simulink model "BLDC_simulator"  (R2024a)
settings: Solver=ode4  StartTime=0.0  StopTime=T  MaxStep=20e-5  RelTol=1e-3  EnableMultiTasking=on
PreLoadFcn:
  | % load scdfocmotorPIDTuning_initial
  | % set_parameters
values from neighbouring files (symbols this model uses):
  current_loop = 1    [BLDC_simulator_init_control.m]    (also in BLDC_simulator_init_control_net_v2_stats_multi.m)
  i_omega = 2.497  * coeff(rand())    [set_parameters_perturbed.m]
  paramPwmCompareAtZeroVolt = 330    [set_parameters_perturbed.m]
  paramPwmCompareMax = 660    [set_parameters_perturbed.m]
  paramPwmComparePerVolt = paramPwmCompareMax/2/BLDC.RatedVoltage    [set_parameters_perturbed.m]
  speed_loop = 1    [BLDC_simulator_init_control.m]    (also in BLDC_simulator_init_control_net_v2_stats_multi.m)
undefined symbols (not defined in the file or in its folder): BLDC, inverter, PID_current, PID_speed, pwm, sampleTime
libraries: nesl_utility x13, fl_lib x12, ee_lib x8, slpidlib x3, simulink x1
(part 2 of 2)

== system BLDC_simulator/Motor_And_Load/Voltage_To_PWM_Compare ==
  note: Voltage To PWM Compare
  Voltage : Inport
  Add : Sum  OutDataTypeStr=Inherit: Inherit via back propagation
  Bias : Constant  Value=paramPwmCompareAtZeroVolt  OutDataTypeStr=Inherit: Inherit via back propagation  SampleTime=-1
  Data_Type_Conversion : DataTypeConversion  OutDataTypeStr=uint16  SaturateOnIntegerOverflow=off  RndMeth=Floor  LockScale=on
  Saturation : Saturate  UpperLimit=paramPwmCompareMax  LowerLimit=0
      settings: AttributesFormatString=|
      | --------------------------------
      | Upper Limit = %<UpperLimit>
      | Lower Limit = %<LowerLimit>
  Slope : Gain  Gain=paramPwmComparePerVolt
      settings: AttributesFormatString=|
      | ----------------------------------------
      | Gain = %<Gain>
  Compare : Outport  VectorParamsAs1DForOutWhenUnconnected=off
  wires:
  Data_Type_Conversion/1 -> Compare/1  "pwmCompare"
  Voltage/1 -> Slope/1  "phaseVoltage"
  Slope/1 -> Add/1
  Saturation/1 -> Data_Type_Conversion/1
  Bias/1 -> Add/2
  Add/1 -> Saturation/1

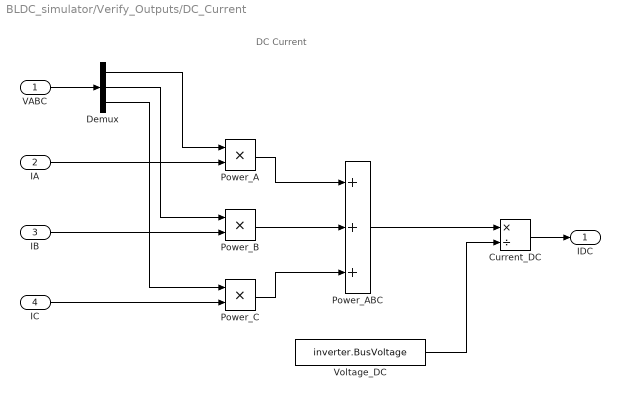
== system BLDC_simulator/Verify_Outputs/DC_Current ==
  note: DC Current
  VABC : Inport
  IA : Inport  Port=2
  IB : Inport  Port=3
  IC : Inport  Port=4
  Current_DC : Product  Inputs=*/
  Demux : Demux  Outputs=3
  Power_A : Product
  Power_ABC : Sum  Inputs=+++
  Power_B : Product
  Power_C : Product
  Voltage_DC : Constant  Value=inverter.BusVoltage
  IDC : Outport  VectorParamsAs1DForOutWhenUnconnected=off
  wires:
  Demux/3 -> Power_C/1
  Demux/2 -> Power_B/1
  Demux/1 -> Power_A/1
  IC/1 -> Power_C/2
  IB/1 -> Power_B/2
  IA/1 -> Power_A/2
  Power_ABC/1 -> Current_DC/1
  Voltage_DC/1 -> Current_DC/2
  Current_DC/1 -> IDC/1
  Power_C/1 -> Power_ABC/3
  VABC/1 -> Demux/1
  Power_B/1 -> Power_ABC/2
  Power_A/1 -> Power_ABC/1

== system BLDC_simulator/Controller_Algorithm/DQ_Current_Control/D_Current_Control ==
  note: D Current Control
  note: D Current Control
  Current_Command : Inport
  Current_Measured : Inport  Port=2
  D current Scope : Scope  NumInputPorts=2
  Error : Sum  Inputs=+-
  PI Controller : slpidlib/PID Controller  Controller=PI  Form=Parallel  TimeDomain=Discrete-time  UseExternalTs=off  SampleTime=sampleTime.CurrentControl  IntegratorMethod=Forward Euler  FilterMethod=Forward Euler  ControllerParametersSource=internal  P=PID_current.p  I=PID_current.i  UseKiTs=off  D=5e-5  UseExternalDerivativeSource=off  N=20000  UseFilter=off  TunerSelectOption=Frequency Response Based  InitialConditionSource=internal  InitialConditionForIntegrator=0  InitialConditionForFilter=0  DifferentiatorICPrevScaledInput=0  ExternalReset=none  TrackingMode=off  Kt=1  LimitOutput=on  SatLimitsSource=internal  UpperSaturationLimit=BLDC.VoltageMax  LowerSaturationLimit=-BLDC.VoltageMax  LinearizeAsGain=off  AntiWindupMode=clamping  Kb=100  LimitIntegrator=off  UpperIntegratorSaturationLimit=inf  LowerIntegratorSaturationLimit=-inf  POutMin=[]  POutMax=[]  IOutMin=[]  IOutMax=[]  DOutMin=[]  DOutMax=[]  NOutMin=[]  NOutMax=[]  SumOutMin=[]  SumOutMax=[]  SaturationOutMin=[]  SaturationOutMax=[]  PParamMin=[]  PParamMax=[]  IParamMin=[]  IParamMax=[]  DParamMin=[]  DParamMax=[]  NParamMin=[]  NParamMax=[]  KbParamMin=[]  KbParamMax=[]  KtParamMin=[]  KtParamMax=[]  KbOutMin=[]  KbOutMax=[]  KtOutMin=[]  KtOutMax=[]  IntegratorOutMin=[]  IntegratorOutMax=[]  FilterOutMin=[]  FilterOutMax=[]  SumI1OutMin=[]  SumI1OutMax=[]  SumI2OutMin=[]  SumI2OutMax=[]  SumI3OutMin=[]  SumI3OutMax=[]  SumI4OutMin=[]  SumI4OutMax=[]  SumDOutMin=[]  SumDOutMax=[]  DifferentiatorOutMin=[]  DifferentiatorOutMax=[]  FilterDiffOutCoefMin=[]  FilterDiffOutCoefMax=[]  ReciprocalOutMin=[]  ReciprocalOutMax=[]  SumDenOutMin=[]  SumDenOutMax=[]  SumNumOutMin=[]  SumNumOutMax=[]  DivideOutMin=[]  DivideOutMax=[]  UdiffTsProdOutMin=[]  UdiffTsProdOutMax=[]  NTsProdOutMin=[]  NTsProdOutMax=[]  UintegralTsProdOutMin=[]  UintegralTsProdOutMax=[]  UngainTsProdOutMin=[]  UngainTsProdOutMax=[]  ClampingZeroOutDataTypeStr=Inherit: Inherit via back propagation  ClampingZeroOutMin=[]  ClampingZeroOutMax=[]  FilterDenConstantOutDataTypeStr=Inherit: Inherit via back propagation  FilterDenConstantOutMin=[]  FilterDenConstantOutMax=[]  PCopyOutDataTypeStr=Inherit: Inherit via back propagation  PCopyOutMin=[]  PCopyOutMax=[]  NCopyOutDataTypeStr=Inherit: Inherit via back propagation  NCopyOutMin=[]  NCopyOutMax=[]  IntegratorContinuousStateAttributes=''  IntegratorStateMustResolveToSignalObject=off  IntegratorRTWStateStorageClass=Auto  FilterContinuousStateAttributes=''  FilterStateMustResolveToSignalObject=off  FilterRTWStateStorageClass=Auto  ParallelPVariant=InternalParameters  IdealPVariant=Disabled  IVariant=InternalParameters  DVariant=Disabled  IntegratorVariant=Discrete  SatVariant=Enabled  AWVariant=DiscClampingParallel  PCopyVariant=Disabled  TRVariant=Disabled  FdbkBlocksVariant=Forward  IdealPFdbkVariant=Disabled  SatFdbkVariant=Disabled  DerivativeFilterVariant=Disabled  NVariant=Disabled  NCopyVariant=Disabled_SignalSpec  FilterICVariant=Disabled  IntegratorICVariant=InternalICs  ExternalResetVariant=Disabled  TRSumVariant=Passthrough  SumFdbkVariant=Disabled  SumVariant=Sum_PI  TsampFilterVariant=InternalTs  TsampNgainVariant=Passthrough  TsampIntegralVariant=Disabled_SignalSpec  ExternalSaturationOutDataTypeStr=Inherit: Same as second input  DerivativeSourceVariant=Disabled
  Voltage : Outport  VectorParamsAs1DForOutWhenUnconnected=off
  wires:
  Error/1 -> PI Controller/1  "currentControlError"
  Current_Command/1 -> Error/1
  PI Controller/1 -> Voltage/1, D current Scope/1  "voltage"
  Current_Measured/1 -> Error/2, D current Scope/2  "current"

== system BLDC_simulator/Controller_Algorithm/DQ_Current_Control/Q_Current_Control ==
  note: Q Current Control
  note: Q Current Control
  Current_Command : Inport
  Current_Measured : Inport  Port=2
  D current Scope : Scope  NumInputPorts=2
  Error : Sum  Inputs=+-
  PI Controller : slpidlib/PID Controller  Controller=PI  Form=Parallel  TimeDomain=Discrete-time  UseExternalTs=off  SampleTime=sampleTime.CurrentControl  IntegratorMethod=Forward Euler  FilterMethod=Forward Euler  ControllerParametersSource=internal  P=PID_current.p  I=PID_current.i  UseKiTs=off  D=5e-5  UseExternalDerivativeSource=off  N=20000  UseFilter=off  TunerSelectOption=Frequency Response Based  InitialConditionSource=internal  InitialConditionForIntegrator=0  InitialConditionForFilter=0  DifferentiatorICPrevScaledInput=0  ExternalReset=none  TrackingMode=off  Kt=1  LimitOutput=on  SatLimitsSource=internal  UpperSaturationLimit=BLDC.VoltageMax  LowerSaturationLimit=-BLDC.VoltageMax  LinearizeAsGain=off  AntiWindupMode=clamping  Kb=100  LimitIntegrator=off  UpperIntegratorSaturationLimit=inf  LowerIntegratorSaturationLimit=-inf  POutMin=[]  POutMax=[]  IOutMin=[]  IOutMax=[]  DOutMin=[]  DOutMax=[]  NOutMin=[]  NOutMax=[]  SumOutMin=[]  SumOutMax=[]  SaturationOutMin=[]  SaturationOutMax=[]  PParamMin=[]  PParamMax=[]  IParamMin=[]  IParamMax=[]  DParamMin=[]  DParamMax=[]  NParamMin=[]  NParamMax=[]  KbParamMin=[]  KbParamMax=[]  KtParamMin=[]  KtParamMax=[]  KbOutMin=[]  KbOutMax=[]  KtOutMin=[]  KtOutMax=[]  IntegratorOutMin=[]  IntegratorOutMax=[]  FilterOutMin=[]  FilterOutMax=[]  SumI1OutMin=[]  SumI1OutMax=[]  SumI2OutMin=[]  SumI2OutMax=[]  SumI3OutMin=[]  SumI3OutMax=[]  SumI4OutMin=[]  SumI4OutMax=[]  SumDOutMin=[]  SumDOutMax=[]  DifferentiatorOutMin=[]  DifferentiatorOutMax=[]  FilterDiffOutCoefMin=[]  FilterDiffOutCoefMax=[]  ReciprocalOutMin=[]  ReciprocalOutMax=[]  SumDenOutMin=[]  SumDenOutMax=[]  SumNumOutMin=[]  SumNumOutMax=[]  DivideOutMin=[]  DivideOutMax=[]  UdiffTsProdOutMin=[]  UdiffTsProdOutMax=[]  NTsProdOutMin=[]  NTsProdOutMax=[]  UintegralTsProdOutMin=[]  UintegralTsProdOutMax=[]  UngainTsProdOutMin=[]  UngainTsProdOutMax=[]  ClampingZeroOutDataTypeStr=Inherit: Inherit via back propagation  ClampingZeroOutMin=[]  ClampingZeroOutMax=[]  FilterDenConstantOutDataTypeStr=Inherit: Inherit via back propagation  FilterDenConstantOutMin=[]  FilterDenConstantOutMax=[]  PCopyOutDataTypeStr=Inherit: Inherit via back propagation  PCopyOutMin=[]  PCopyOutMax=[]  NCopyOutDataTypeStr=Inherit: Inherit via back propagation  NCopyOutMin=[]  NCopyOutMax=[]  IntegratorContinuousStateAttributes=''  IntegratorStateMustResolveToSignalObject=off  IntegratorRTWStateStorageClass=Auto  FilterContinuousStateAttributes=''  FilterStateMustResolveToSignalObject=off  FilterRTWStateStorageClass=Auto  ParallelPVariant=InternalParameters  IdealPVariant=Disabled  IVariant=InternalParameters  DVariant=Disabled  IntegratorVariant=Discrete  SatVariant=Enabled  AWVariant=DiscClampingParallel  PCopyVariant=Disabled  TRVariant=Disabled  FdbkBlocksVariant=Forward  IdealPFdbkVariant=Disabled  SatFdbkVariant=Disabled  DerivativeFilterVariant=Disabled  NVariant=Disabled  NCopyVariant=Disabled_SignalSpec  FilterICVariant=Disabled  IntegratorICVariant=InternalICs  ExternalResetVariant=Disabled  TRSumVariant=Passthrough  SumFdbkVariant=Disabled  SumVariant=Sum_PI  TsampFilterVariant=InternalTs  TsampNgainVariant=Passthrough  TsampIntegralVariant=Disabled_SignalSpec  ExternalSaturationOutDataTypeStr=Inherit: Same as second input  DerivativeSourceVariant=Disabled
  Voltage : Outport  VectorParamsAs1DForOutWhenUnconnected=off
  wires:
  Error/1 -> PI Controller/1  "currentControlError"
  Current_Command/1 -> Error/1
  PI Controller/1 -> Voltage/1, D current Scope/1  "voltage"
  Current_Measured/1 -> Error/2, D current Scope/2  "current"

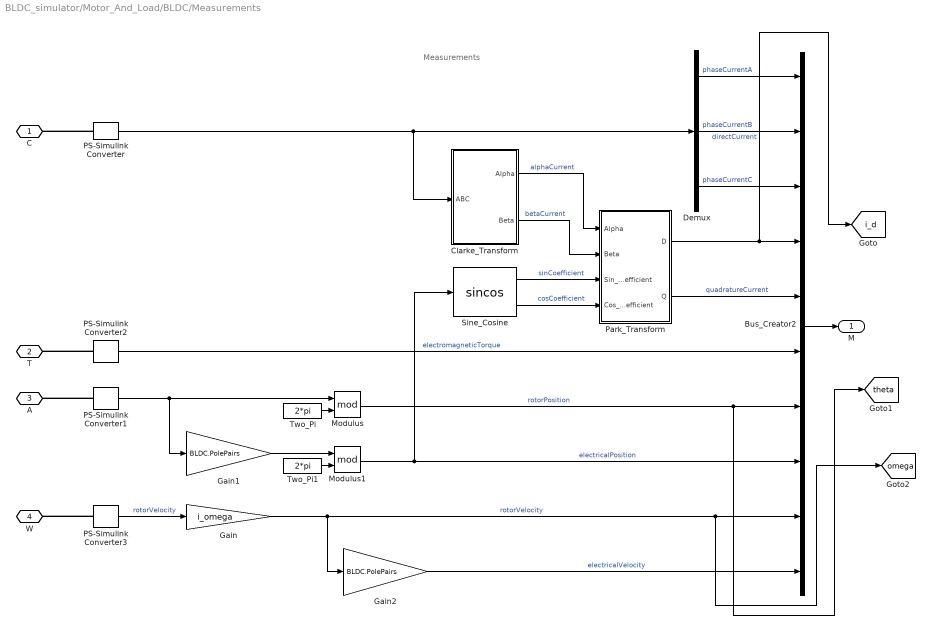
== system BLDC_simulator/Motor_And_Load/BLDC/Measurements ==
  note: Measurements
  Bus_Creator2 : BusCreator  Inputs=10
  Clarke_Transform : Subsystem
      mask Display:
      | port_label('input',1,'ABC')
      | port_label('output',1,'\alpha','texmode', 'on')
      | port_label('output',2,'\beta','texmode', 'on')
  Demux : Demux  Outputs=3
  Gain : Gain  Gain=i_omega
  Gain1 : Gain  Gain=BLDC.PolePairs
      settings: AttributesFormatString=-----------------------------\n%<Gain>
  Gain2 : Gain  Gain=BLDC.PolePairs
      settings: AttributesFormatString=-----------------------------\n%<Gain>
  Modulus : Math  Operator=mod  SignedPower=on
  Modulus1 : Math  Operator=mod  SignedPower=on
  PS-Simulink Converter : nesl_utility/PS-Simulink Converter  PhysicalDomain=network_engine_domain  SubClassName=ps_output  LeftPortType=input  RightPortType=output  PseudoPeriodic=off  Frequencies=[]  VectorFormat=1-D array  Unit=A  AffineConversion=off
  PS-Simulink Converter1 : nesl_utility/PS-Simulink Converter  PhysicalDomain=network_engine_domain  SubClassName=ps_output  LeftPortType=input  RightPortType=output  PseudoPeriodic=off  Frequencies=[]  VectorFormat=1-D array  Unit=rad  AffineConversion=off
  PS-Simulink Converter2 : nesl_utility/PS-Simulink Converter  PhysicalDomain=network_engine_domain  SubClassName=ps_output  LeftPortType=input  RightPortType=output  PseudoPeriodic=off  Frequencies=[]  VectorFormat=1-D array  Unit=N*m  AffineConversion=off
  PS-Simulink Converter3 : nesl_utility/PS-Simulink Converter  PhysicalDomain=network_engine_domain  SubClassName=ps_output  LeftPortType=input  RightPortType=output  PseudoPeriodic=off  Frequencies=[]  VectorFormat=1-D array  Unit=rad/s  AffineConversion=off
  Park_Transform : Subsystem
      mask Display:
      | port_label('input',1,'\alpha','texmode', 'on')
      | port_label('input',2,'\beta','texmode', 'on')
      | port_label('input',3,'Sin')
      | port_label('input',4,'Cos')
      | port_label('output',1,'D')
      | port_label('output',2,'Q')
  Sine_Cosine : Trigonometry  Operator=sincos
  Two_Pi : Constant  Value=2*pi  OutDataTypeStr=Inherit: Inherit via back propagation
  Two_Pi1 : Constant  Value=2*pi  OutDataTypeStr=Inherit: Inherit via back propagation
  C : PMIOPort  Side=Left
  T : PMIOPort  Port=2  Side=Left
  A : PMIOPort  Port=3  Side=Left
  W : PMIOPort  Port=4  Side=Left
  M : Outport  VectorParamsAs1DForOutWhenUnconnected=off
  tag scope: i_d=global, omega=global, theta=global
  wires:
  Demux/2 -> Bus_Creator2/2  "phaseCurrentB"
  Demux/3 -> Bus_Creator2/3  "phaseCurrentC"
  Demux/1 -> Bus_Creator2/1  "phaseCurrentA"
  PS-Simulink Converter/1 -> Clarke_Transform/1(ABC), Demux/1
  Bus_Creator2/1 -> M/1
  PS-Simulink Converter2/1 -> Bus_Creator2/6  "electromagneticTorque"
  PS-Simulink Converter3/1 -> Gain/1  "rotorVelocity"
  Modulus/1 -> [theta], Bus_Creator2/7  "rotorPosition"
  Modulus1/1 -> Sine_Cosine/1, Bus_Creator2/8  "electricalPosition"
  Gain2/1 -> Bus_Creator2/10  "electricalVelocity"
  Two_Pi/1 -> Modulus/2
  Two_Pi1/1 -> Modulus1/2
  Gain1/1 -> Modulus1/1
  PS-Simulink Converter1/1 -> Modulus/1, Gain1/1
  Sine_Cosine/1 -> Park_Transform/3(Sin_Coefficient)  "sinCoefficient"
  Sine_Cosine/2 -> Park_Transform/4(Cos_Coefficient)  "cosCoefficient"
  Clarke_Transform/2(Beta) -> Park_Transform/2(Beta)  "betaCurrent"
  Clarke_Transform/1(Alpha) -> Park_Transform/1(Alpha)  "alphaCurrent"
  Park_Transform/1(D) -> [i_d], Bus_Creator2/4  "directCurrent"
  Park_Transform/2(Q) -> Bus_Creator2/5  "quadratureCurrent"
  Gain/1 -> [omega], Bus_Creator2/9, Gain2/1  "rotorVelocity"
  connections:
  PS-Simulink Converter/LConn1 -- C/RConn1
  PS-Simulink Converter1/LConn1 -- A/RConn1
  PS-Simulink Converter2/LConn1 -- T/RConn1
  PS-Simulink Converter3/LConn1 -- W/RConn1

== system BLDC_simulator/Motor_And_Load/BLDC/Measurements/Clarke_Transform ==
  note: Clarke Transform
  ABC : Inport
  A : Selector  IndexMode=Zero-based  InputPortWidth=3  IndexOptions=Index vector (dialog)  Indices=0  OutputSizes=1
  Add : Sum  OutDataTypeStr=Inherit: Same as first input
  Alpha_Gain : Gain  Gain=1/sqrt(3)
  B : Selector  IndexMode=Zero-based  InputPortWidth=3  IndexOptions=Index vector (dialog)  Indices=1  OutputSizes=1
  Beta_Gain : Gain  Gain=2/sqrt(3)
  Alpha : Outport  VectorParamsAs1DForOutWhenUnconnected=off
  Beta : Outport  Port=2  VectorParamsAs1DForOutWhenUnconnected=off
  wires:
  Add/1 -> Beta/1
  B/1 -> Beta_Gain/1
  Beta_Gain/1 -> Add/2
  ABC/1 -> A/1, B/1
  Alpha_Gain/1 -> Add/1
  A/1 -> Alpha_Gain/1, Alpha/1

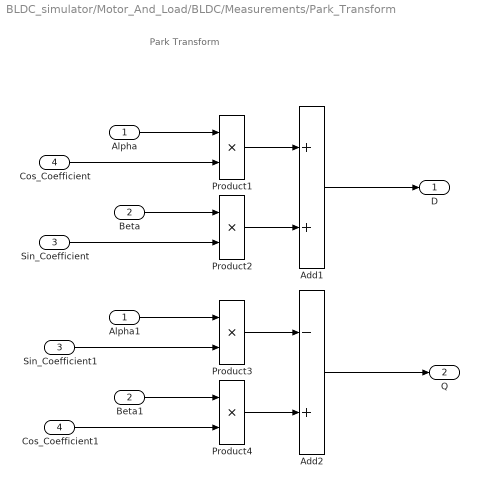
== system BLDC_simulator/Motor_And_Load/BLDC/Measurements/Park_Transform ==
  note: Park Transform
  Alpha : Inport
  Beta : Inport  Port=2
  Sin_Coefficient : Inport  Port=3
  Cos_Coefficient : Inport  Port=4
  Add1 : Sum  OutDataTypeStr=Inherit: Same as first input
  Add2 : Sum  Inputs=-+  OutDataTypeStr=Inherit: Same as first input
  Alpha1 : InportShadow
  Beta1 : InportShadow  Port=2
  Cos_Coefficient1 : InportShadow  Port=4
  Product{1..4} (4 alike) : Product  RndMeth=Simplest
  Sin_Coefficient1 : InportShadow  Port=3
  D : Outport  VectorParamsAs1DForOutWhenUnconnected=off
  Q : Outport  Port=2  VectorParamsAs1DForOutWhenUnconnected=off
  wires:
  Product3/1 -> Add2/1
  Product4/1 -> Add2/2
  Product1/1 -> Add1/1
  Product2/1 -> Add1/2
  Alpha1/1 -> Product3/1
  Sin_Coefficient1/1 -> Product3/2
  Cos_Coefficient1/1 -> Product4/2
  Beta1/1 -> Product4/1
  Alpha/1 -> Product1/1
  Cos_Coefficient/1 -> Product1/2
  Beta/1 -> Product2/1
  Sin_Coefficient/1 -> Product2/2
  Add1/1 -> D/1
  Add2/1 -> Q/1
